simulink model "tb_rc_sbus_encoder"  (R2026b)
values from neighbouring files (symbols this model uses):
  Ts = prm.Ts    [row_driver_bench.m]
libraries: simulink x1
settings Model: Creator=aomar  LastModifiedBy=aomar

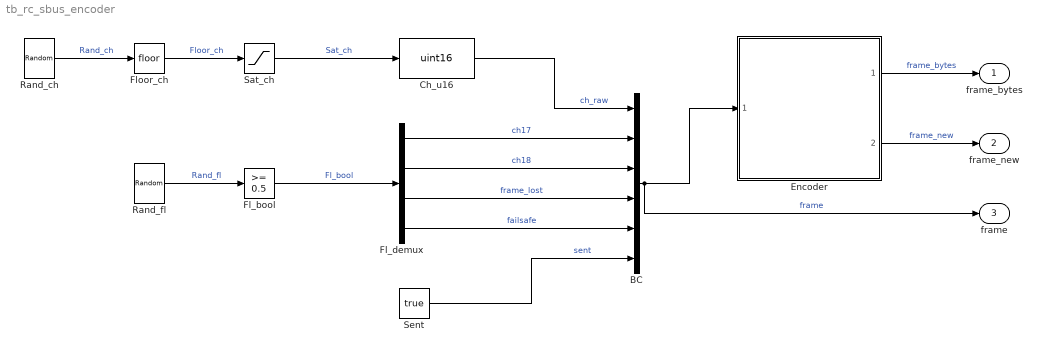
== system tb_rc_sbus_encoder ==
  BC : BusCreator  Inputs=6  OutDataTypeStr=Bus: Bus_RcFrame  NonVirtualBus=on
      settings: InheritFromInputs=off
  Ch_u16 : DataTypeConversion  OutDataTypeStr=uint16  SaturateOnIntegerOverflow=off  RndMeth=Floor
  Encoder : Subsystem  ReferencedSubsystem=rc_sbus_encoder
  Fl_bool : simulink/Logic and Bit Operations/Compare To Constant  relop=>=  const=0.5  OutDataTypeStr=boolean
  Fl_demux : Demux
  Floor_ch : Rounding
  Rand_ch : UniformRandomNumber  Minimum=zeros(1,16)  Maximum=2048*ones(1,16)  Seed=7*(1:16)+11  SampleTime=Ts.rc_frame
  Rand_fl : UniformRandomNumber  Minimum=zeros(1,4)  Maximum=ones(1,4)  Seed=101:104  SampleTime=Ts.rc_frame
  Sat_ch : Saturate  UpperLimit=2047  LowerLimit=0
  Sent : Constant  Value=true  OutDataTypeStr=boolean  SampleTime=Ts.rc_frame
  frame_bytes : Outport  OutDataTypeStr=uint8
  frame_new : Outport  Port=2  OutDataTypeStr=boolean
  frame : Outport  Port=3  OutDataTypeStr=Bus: Bus_RcFrame
  wires:
  Rand_ch/1 -> Floor_ch/1  "Rand_ch"
  Floor_ch/1 -> Sat_ch/1  "Floor_ch"
  Rand_fl/1 -> Fl_bool/1  "Rand_fl"
  Sat_ch/1 -> Ch_u16/1  "Sat_ch"
  Fl_bool/1 -> Fl_demux/1  "Fl_bool"
  Fl_demux/1 -> BC/2  "ch17"
  Fl_demux/2 -> BC/3  "ch18"
  Fl_demux/3 -> BC/4  "frame_lost"
  Fl_demux/4 -> BC/5  "failsafe"
  Sent/1 -> BC/6  "sent"
  Ch_u16/1 -> BC/1  "ch_raw"
  BC/1 -> Encoder/1, frame/1  "frame"
  Encoder/1 -> frame_bytes/1  "frame_bytes"
  Encoder/2 -> frame_new/1  "frame_new"
